simulink model "sm_car_"  (R2026b)
settings: Solver=ode23t  StopTime=100  MaxStep=0.4  AbsTol=1e-3  EnableMultiTasking=on
PreLoadFcn:
  | % Due to usability issue in Repeating Sequence block
  | warning('off','Simulink:Masking:Invalid');
  | 
  | % Eliminate unnecessary warnings in inactive variants
  | % Warnings generated only if you click through inactive variant
  | warning('off','MATLAB:nonExistentField');
  | warning('off','Simulink:Parameters:BlkParamUndefined');
PostLoadFcn:
  | set_param([bdroot '/Vehicle'],'popup_trailer','Off')
  | warning('off','sm:sli:setup:compile:LocalSolverNotSupported')
  | %sm_car_config_maneuver(bdroot,'WOT Braking');
  | sm_car_config_vehicle(bdroot,'false');
  | sm_car_config_logging(bdroot);
InitFcn:
  | sm_car_config_camera;
  | Vehicle = sm_car_vehcfg_checkConfig(Vehicle);
  | sm_car_check_tire_model(bdroot);
StartFcn:
  | tic;
StopFcn:
  | Elapsed_Sim_Time = toc;
  | % disp(['Elapsed Sim Time = ' num2str(Elapsed_Sim_Time)]);
undefined symbols (not defined in the file or in its folder): acc_theta, accel_ramp_rate, Axle1D, AxleIn, Camera, Control, Driver, Init, Maneuver, Pedal, Scene, ShaftL1, ShaftL2, ShaftR1, ShaftR2, Visual, X, xy_data_car_side, Y, Z
libraries: sm_lib x290, fl_lib x171, nesl_utility x144, simulink x60, simulink_extras x14, sdl_lib x14, SimscapeFluids_lib x7, Damper_Element x4, Tire_1x2x x4, ee_lib x3, Scene_Utilities x3, sharedTrackingLibrary x2
(part 21 of 22)

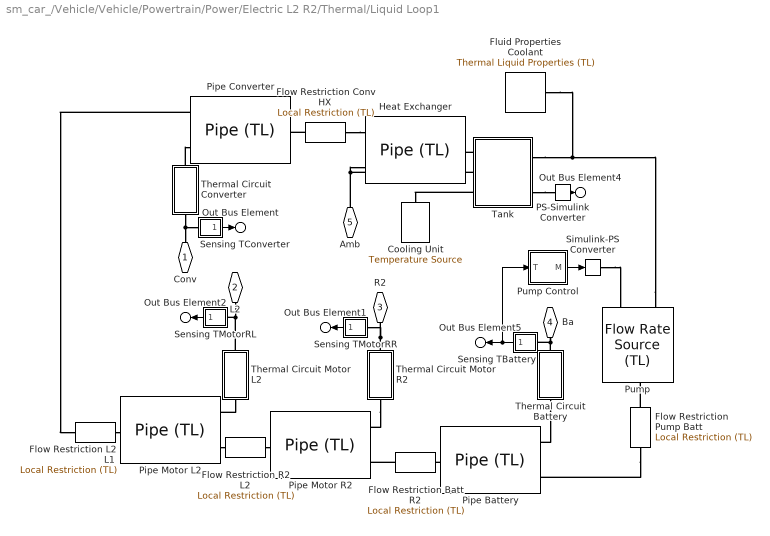
== system sm_car_/Vehicle/Vehicle/Powertrain/Power/Electric L2 R2/Thermal/Liquid Loop1 ==
  Cooling Unit : fl_lib/Thermal/Thermal Sources/Temperature Source  temperature=278 K
  Flow Restriction Batt R2 : fl_lib/Thermal Liquid/Elements/Local Restriction (TL)  restriction_type=foundation.enum.restriction_type.fixed  restriction_area=0.01^2/4*pi*0.5 m^2  min_area=1e-10 m^2  max_area=0.005 m^2  area=0.01^2/4*pi m^2  Cd=0.7  Re_c=12  pressure_recovery=1
  Flow Restriction Conv HX : fl_lib/Thermal Liquid/Elements/Local Restriction (TL)  restriction_type=foundation.enum.restriction_type.fixed  restriction_area=0.01^2/4*pi*0.5 m^2  min_area=1e-10 m^2  max_area=0.005 m^2  area=0.01^2/4*pi m^2  Cd=0.7  Re_c=12  pressure_recovery=1
  Flow Restriction L2 L1 : fl_lib/Thermal Liquid/Elements/Local Restriction (TL)  restriction_type=foundation.enum.restriction_type.fixed  restriction_area=0.01^2/4*pi*0.5 m^2  min_area=1e-10 m^2  max_area=0.005 m^2  area=0.01^2/4*pi m^2  Cd=0.7  Re_c=12  pressure_recovery=1
  Flow Restriction Pump Batt : fl_lib/Thermal Liquid/Elements/Local Restriction (TL)  restriction_type=foundation.enum.restriction_type.fixed  restriction_area=0.01^2/4*pi*0.5 m^2  min_area=1e-10 m^2  max_area=0.005 m^2  area=0.01^2/4*pi m^2  Cd=0.7  Re_c=12  pressure_recovery=1
  Flow Restriction R2 L2 : fl_lib/Thermal Liquid/Elements/Local Restriction (TL)  restriction_type=foundation.enum.restriction_type.fixed  restriction_area=0.01^2/4*pi*0.5 m^2  min_area=1e-10 m^2  max_area=0.005 m^2  area=0.01^2/4*pi m^2  Cd=0.7  Re_c=12  pressure_recovery=1
  "Fluid Properties Coolant " : SimscapeFluids_lib/Thermal Liquid/Utilities/Thermal Liquid Properties (TL)  fluid_list=fluids.thermal_liquid.utilities.enum.thermal_liquid_fluid_list.ethylene_glycol  concentration_param_EG=fluids.thermal_liquid.utilities.enum.thermal_liquid_concentration.volume_fraction  concentration_param_PG=fluids.thermal_liquid.utilities.enum.thermal_liquid_concentration.volume_fraction  c_mass_SW=3.5e-3  c_mass_EG=0.1  c_mass_PG=0.1  c_mass_GL=0.1  c_vol_EG=0.1  c_vol_PG=0.1  beta_const_EG=2.1791 GPa  beta_const_PG=2.1791 GPa  beta_const_GL=2.1791 GPa  p_min_EG=0.01 MPa  p_min_PG=0.01 MPa  p_min_GL=0.01 MPa  p_max_EG=50 MPa  p_max_PG=50 MPa  p_max_GL=50 MPa  T_atm=293.15 K  p_atm=0.101325 MPa  properties_range_check=simscape.enum.assert.action.error  air_fraction=0  R_air=0.287 kJ/(K*kg)  air_dissolution_model=false  p_crit=3 MPa
  Heat Exchanger : SimscapeFluids_lib/Thermal Liquid/Pipes & Fittings/Pipe (TL)  dynamic_compressibility=0  inertia=0  num_segments=1  pipe_length=10 m  cross_section_geometry=fluids.thermal_liquid.pipes_fittings.enum.CrossSectionGeometry.Custom  pipe_diameter=0.1 m  pipe_inner_diameter=0.05 m  pipe_outer_diameter=0.1 m  pipe_width=0.1 m  pipe_height=0.1 m  pipe_major_axis=0.1 m  pipe_minor_axis=0.05 m  pipe_side=0.1 m  pipe_angle=30 deg  area=0.01^2/4*pi m^2  Dh=0.1128 m  annular_heat_transfer_walls=fluids.thermal_liquid.pipes_fittings.enum.AnnularPipeWalls.AnnularInner  elevation_spec=foundation.enum.constant_variable.constant  elevation_gain=0 m  gravity_spec=foundation.enum.constant_variable.constant  g=9.81 m/s^2  pressure_loss_spec=1  local_pressure_loss_spec=fluids.thermal_liquid.pipes_fittings.enum.LocalLossSpec.AggregateLength  length_add=0.1 m  loss_coefficient=0.1  roughness_spec=fluids.thermal_liquid.pipes_fittings.enum.RoughnessSpec.Custom  roughness=1.5e-5 m  Re_friction_TLU=[ 400 1000 1.5e+3 3e+3 4e+3 6e+3 1e+4 2e+4 4e+4 6e+4 1e+5 1e+8 ]  friction_factor_TLU=[ 0.264 0.112 0.07099999999999999 0.0417 0.0387 0.0268 0.025 0.0232 0.0226 0.022 0.0214 0.0214 ]  Re_lam=2e+3  Re_tur=4e+3  shape_factor=64  mdot_nominal=[ 0.1 1 ] kg/s  p_diff_nominal=[ 0.001 0.01 ] MPa  mdot_threshold=1e-6 kg/s  wall_spec=1  vol_expansion_spec=fluids.thermal_liquid.pipes_fittings.enum.VolumeExpansionSpec.Diameter  area_pressure_gain=1e-6 m^2/MPa  static_pressure_TLU=[.1, 1] MPa  area_pressure_gain_TLU=[1e-05, 1.1e-05] m^2  material_behavior_spec=fluids.thermal_liquid.pipes_fittings.enum.PipeMaterialBehavior.Linear  diameter_pressure_gain=1.2e-6 m/MPa  wall_thickness=0.05 m  elastic_modulus=69 GPa  stress_TLU=[276, 310] MPa  strain_TLU=[.004, .02]  stress_assert_action=simscape.enum.assert.action.none  stress_max=400 MPa  poisson_ratio=0.33  wall_time_constant=0.01 s  environment_spec=foundation.enum.pressure_spec.atmospheric  environment_pressure=0.101325 MPa  thermal_expansion=false  alpha_L_wall=24 um/(deltaK*m)  thermal_expansion_Tref=293.15 K  heat_transfer_spec=1  mdot_nominal_heat=[ 0.1 1 ] kg/s  T_in_nominal=[ 293.15 293.15 ] K  T_out_nominal=[ 300 300 ] K  p_in_nominal_heat=[ 0.101325 0.101325 ] MPa  T_wall_nominal=[ 303.15 303.15 ] K  T_wall_eff_nominal=[303.15, 303.15] K  a_coeff=0.023  b_Re_power=0.8  c_Pr_power=0.4  Nu_lam=3.66  Re_Colburn_TLU=[ 100 150 1000 ]  Colburn_factor_TLU=[ 0.019 0.013 0.002 ]  Re_Nu_TLU=[ 100 150 1000 ]  Pr_Nu_TLU=[ 1 10 ]  Nu_TLU=[ 3.72 4.21; 3.75 4.44; 4.21 7.15 ]  annular_correction=fluids.thermal_liquid.pipes_fittings.enum.AnnularPipeCorrectionFactor.Gnielinski  p0_vec=0.101325 MPa  T0_vec=300 K  mdot0=0.1 kg/s  p_nominal=0.101325 MPa  T_nominal=293.15 K
  PS-Simulink Converter : nesl_utility/PS-Simulink Converter  PhysicalDomain=network_engine_domain  SubClassName=ps_output  LeftPortType=input  RightPortType=output  PseudoPeriodic=off  Frequencies=[]  VectorFormat=1-D array  Unit=1  AffineConversion=off
  Pipe Battery : SimscapeFluids_lib/Thermal Liquid/Pipes & Fittings/Pipe (TL)  dynamic_compressibility=0  inertia=0  num_segments=1  pipe_length=1 m  cross_section_geometry=fluids.thermal_liquid.pipes_fittings.enum.CrossSectionGeometry.Custom  pipe_diameter=0.1 m  pipe_inner_diameter=0.05 m  pipe_outer_diameter=0.1 m  pipe_width=0.1 m  pipe_height=0.1 m  pipe_major_axis=0.1 m  pipe_minor_axis=0.05 m  pipe_side=0.1 m  pipe_angle=30 deg  area=0.01^2/4*pi m^2  Dh=0.1128 m  annular_heat_transfer_walls=fluids.thermal_liquid.pipes_fittings.enum.AnnularPipeWalls.AnnularInner  elevation_spec=foundation.enum.constant_variable.constant  elevation_gain=0 m  gravity_spec=foundation.enum.constant_variable.constant  g=9.81 m/s^2  pressure_loss_spec=1  local_pressure_loss_spec=fluids.thermal_liquid.pipes_fittings.enum.LocalLossSpec.AggregateLength  length_add=0.1 m  loss_coefficient=0.1  roughness_spec=fluids.thermal_liquid.pipes_fittings.enum.RoughnessSpec.Custom  roughness=1.5e-5 m  Re_friction_TLU=[ 400 1000 1.5e+3 3e+3 4e+3 6e+3 1e+4 2e+4 4e+4 6e+4 1e+5 1e+8 ]  friction_factor_TLU=[ 0.264 0.112 0.07099999999999999 0.0417 0.0387 0.0268 0.025 0.0232 0.0226 0.022 0.0214 0.0214 ]  Re_lam=2e+3  Re_tur=4e+3  shape_factor=64  mdot_nominal=[ 0.1 1 ] kg/s  p_diff_nominal=[ 0.001 0.01 ] MPa  mdot_threshold=1e-6 kg/s  wall_spec=1  vol_expansion_spec=fluids.thermal_liquid.pipes_fittings.enum.VolumeExpansionSpec.Diameter  area_pressure_gain=1e-6 m^2/MPa  static_pressure_TLU=[.1, 1] MPa  area_pressure_gain_TLU=[1e-05, 1.1e-05] m^2  material_behavior_spec=fluids.thermal_liquid.pipes_fittings.enum.PipeMaterialBehavior.Linear  diameter_pressure_gain=1.2e-6 m/MPa  wall_thickness=0.05 m  elastic_modulus=69 GPa  stress_TLU=[276, 310] MPa  strain_TLU=[.004, .02]  stress_assert_action=simscape.enum.assert.action.none  stress_max=400 MPa  poisson_ratio=0.33  wall_time_constant=0.01 s  environment_spec=foundation.enum.pressure_spec.atmospheric  environment_pressure=0.101325 MPa  thermal_expansion=false  alpha_L_wall=24 um/(deltaK*m)  thermal_expansion_Tref=293.15 K  heat_transfer_spec=1  mdot_nominal_heat=[ 0.1 1 ] kg/s  T_in_nominal=[ 293.15 293.15 ] K  T_out_nominal=[ 300 300 ] K  p_in_nominal_heat=[ 0.101325 0.101325 ] MPa  T_wall_nominal=[ 303.15 303.15 ] K  T_wall_eff_nominal=[303.15, 303.15] K  a_coeff=0.023  b_Re_power=0.8  c_Pr_power=0.4  Nu_lam=3.66  Re_Colburn_TLU=[ 100 150 1000 ]  Colburn_factor_TLU=[ 0.019 0.013 0.002 ]  Re_Nu_TLU=[ 100 150 1000 ]  Pr_Nu_TLU=[ 1 10 ]  Nu_TLU=[ 3.72 4.21; 3.75 4.44; 4.21 7.15 ]  annular_correction=fluids.thermal_liquid.pipes_fittings.enum.AnnularPipeCorrectionFactor.Gnielinski  p0_vec=0.101325 MPa  T0_vec=300 K  mdot0=0.1 kg/s  p_nominal=0.101325 MPa  T_nominal=293.15 K
  Pipe Converter : SimscapeFluids_lib/Thermal Liquid/Pipes & Fittings/Pipe (TL)  dynamic_compressibility=0  inertia=0  num_segments=1  pipe_length=1 m  cross_section_geometry=fluids.thermal_liquid.pipes_fittings.enum.CrossSectionGeometry.Custom  pipe_diameter=0.1 m  pipe_inner_diameter=0.05 m  pipe_outer_diameter=0.1 m  pipe_width=0.1 m  pipe_height=0.1 m  pipe_major_axis=0.1 m  pipe_minor_axis=0.05 m  pipe_side=0.1 m  pipe_angle=30 deg  area=0.01^2/4*pi m^2  Dh=0.1128 m  annular_heat_transfer_walls=fluids.thermal_liquid.pipes_fittings.enum.AnnularPipeWalls.AnnularInner  elevation_spec=foundation.enum.constant_variable.constant  elevation_gain=0 m  gravity_spec=foundation.enum.constant_variable.constant  g=9.81 m/s^2  pressure_loss_spec=1  local_pressure_loss_spec=fluids.thermal_liquid.pipes_fittings.enum.LocalLossSpec.AggregateLength  length_add=0.1 m  loss_coefficient=0.1  roughness_spec=fluids.thermal_liquid.pipes_fittings.enum.RoughnessSpec.Custom  roughness=1.5e-5 m  Re_friction_TLU=[ 400 1000 1.5e+3 3e+3 4e+3 6e+3 1e+4 2e+4 4e+4 6e+4 1e+5 1e+8 ]  friction_factor_TLU=[ 0.264 0.112 0.07099999999999999 0.0417 0.0387 0.0268 0.025 0.0232 0.0226 0.022 0.0214 0.0214 ]  Re_lam=2e+3  Re_tur=4e+3  shape_factor=64  mdot_nominal=[ 0.1 1 ] kg/s  p_diff_nominal=[ 0.001 0.01 ] MPa  mdot_threshold=1e-6 kg/s  wall_spec=1  vol_expansion_spec=fluids.thermal_liquid.pipes_fittings.enum.VolumeExpansionSpec.Diameter  area_pressure_gain=1e-6 m^2/MPa  static_pressure_TLU=[.1, 1] MPa  area_pressure_gain_TLU=[1e-05, 1.1e-05] m^2  material_behavior_spec=fluids.thermal_liquid.pipes_fittings.enum.PipeMaterialBehavior.Linear  diameter_pressure_gain=1.2e-6 m/MPa  wall_thickness=0.05 m  elastic_modulus=69 GPa  stress_TLU=[276, 310] MPa  strain_TLU=[.004, .02]  stress_assert_action=simscape.enum.assert.action.none  stress_max=400 MPa  poisson_ratio=0.33  wall_time_constant=0.01 s  environment_spec=foundation.enum.pressure_spec.atmospheric  environment_pressure=0.101325 MPa  thermal_expansion=false  alpha_L_wall=24 um/(deltaK*m)  thermal_expansion_Tref=293.15 K  heat_transfer_spec=1  mdot_nominal_heat=[ 0.1 1 ] kg/s  T_in_nominal=[ 293.15 293.15 ] K  T_out_nominal=[ 300 300 ] K  p_in_nominal_heat=[ 0.101325 0.101325 ] MPa  T_wall_nominal=[ 303.15 303.15 ] K  T_wall_eff_nominal=[303.15, 303.15] K  a_coeff=0.023  b_Re_power=0.8  c_Pr_power=0.4  Nu_lam=3.66  Re_Colburn_TLU=[ 100 150 1000 ]  Colburn_factor_TLU=[ 0.019 0.013 0.002 ]  Re_Nu_TLU=[ 100 150 1000 ]  Pr_Nu_TLU=[ 1 10 ]  Nu_TLU=[ 3.72 4.21; 3.75 4.44; 4.21 7.15 ]  annular_correction=fluids.thermal_liquid.pipes_fittings.enum.AnnularPipeCorrectionFactor.Gnielinski  p0_vec=0.101325 MPa  T0_vec=300 K  mdot0=0.1 kg/s  p_nominal=0.101325 MPa  T_nominal=293.15 K
  Pipe Motor L2 : SimscapeFluids_lib/Thermal Liquid/Pipes & Fittings/Pipe (TL)  dynamic_compressibility=0  inertia=0  num_segments=1  pipe_length=1 m  cross_section_geometry=fluids.thermal_liquid.pipes_fittings.enum.CrossSectionGeometry.Custom  pipe_diameter=0.1 m  pipe_inner_diameter=0.05 m  pipe_outer_diameter=0.1 m  pipe_width=0.1 m  pipe_height=0.1 m  pipe_major_axis=0.1 m  pipe_minor_axis=0.05 m  pipe_side=0.1 m  pipe_angle=30 deg  area=0.01^2/4*pi m^2  Dh=0.1128 m  annular_heat_transfer_walls=fluids.thermal_liquid.pipes_fittings.enum.AnnularPipeWalls.AnnularInner  elevation_spec=foundation.enum.constant_variable.constant  elevation_gain=0 m  gravity_spec=foundation.enum.constant_variable.constant  g=9.81 m/s^2  pressure_loss_spec=1  local_pressure_loss_spec=fluids.thermal_liquid.pipes_fittings.enum.LocalLossSpec.AggregateLength  length_add=0.1 m  loss_coefficient=0.1  roughness_spec=fluids.thermal_liquid.pipes_fittings.enum.RoughnessSpec.Custom  roughness=1.5e-5 m  Re_friction_TLU=[ 400 1000 1.5e+3 3e+3 4e+3 6e+3 1e+4 2e+4 4e+4 6e+4 1e+5 1e+8 ]  friction_factor_TLU=[ 0.264 0.112 0.07099999999999999 0.0417 0.0387 0.0268 0.025 0.0232 0.0226 0.022 0.0214 0.0214 ]  Re_lam=2e+3  Re_tur=4e+3  shape_factor=64  mdot_nominal=[ 0.1 1 ] kg/s  p_diff_nominal=[ 0.001 0.01 ] MPa  mdot_threshold=1e-6 kg/s  wall_spec=1  vol_expansion_spec=fluids.thermal_liquid.pipes_fittings.enum.VolumeExpansionSpec.Diameter  area_pressure_gain=1e-6 m^2/MPa  static_pressure_TLU=[.1, 1] MPa  area_pressure_gain_TLU=[1e-05, 1.1e-05] m^2  material_behavior_spec=fluids.thermal_liquid.pipes_fittings.enum.PipeMaterialBehavior.Linear  diameter_pressure_gain=1.2e-6 m/MPa  wall_thickness=0.05 m  elastic_modulus=69 GPa  stress_TLU=[276, 310] MPa  strain_TLU=[.004, .02]  stress_assert_action=simscape.enum.assert.action.none  stress_max=400 MPa  poisson_ratio=0.33  wall_time_constant=0.01 s  environment_spec=foundation.enum.pressure_spec.atmospheric  environment_pressure=0.101325 MPa  thermal_expansion=false  alpha_L_wall=24 um/(deltaK*m)  thermal_expansion_Tref=293.15 K  heat_transfer_spec=1  mdot_nominal_heat=[ 0.1 1 ] kg/s  T_in_nominal=[ 293.15 293.15 ] K  T_out_nominal=[ 300 300 ] K  p_in_nominal_heat=[ 0.101325 0.101325 ] MPa  T_wall_nominal=[ 303.15 303.15 ] K  T_wall_eff_nominal=[303.15, 303.15] K  a_coeff=0.023  b_Re_power=0.8  c_Pr_power=0.4  Nu_lam=3.66  Re_Colburn_TLU=[ 100 150 1000 ]  Colburn_factor_TLU=[ 0.019 0.013 0.002 ]  Re_Nu_TLU=[ 100 150 1000 ]  Pr_Nu_TLU=[ 1 10 ]  Nu_TLU=[ 3.72 4.21; 3.75 4.44; 4.21 7.15 ]  annular_correction=fluids.thermal_liquid.pipes_fittings.enum.AnnularPipeCorrectionFactor.Gnielinski  p0_vec=0.101325 MPa  T0_vec=300 K  mdot0=0.1 kg/s  p_nominal=0.101325 MPa  T_nominal=293.15 K
  Pipe Motor R2 : SimscapeFluids_lib/Thermal Liquid/Pipes & Fittings/Pipe (TL)  dynamic_compressibility=0  inertia=0  num_segments=1  pipe_length=1 m  cross_section_geometry=fluids.thermal_liquid.pipes_fittings.enum.CrossSectionGeometry.Custom  pipe_diameter=0.1 m  pipe_inner_diameter=0.05 m  pipe_outer_diameter=0.1 m  pipe_width=0.1 m  pipe_height=0.1 m  pipe_major_axis=0.1 m  pipe_minor_axis=0.05 m  pipe_side=0.1 m  pipe_angle=30 deg  area=0.01^2/4*pi m^2  Dh=0.1128 m  annular_heat_transfer_walls=fluids.thermal_liquid.pipes_fittings.enum.AnnularPipeWalls.AnnularInner  elevation_spec=foundation.enum.constant_variable.constant  elevation_gain=0 m  gravity_spec=foundation.enum.constant_variable.constant  g=9.81 m/s^2  pressure_loss_spec=1  local_pressure_loss_spec=fluids.thermal_liquid.pipes_fittings.enum.LocalLossSpec.AggregateLength  length_add=0.1 m  loss_coefficient=0.1  roughness_spec=fluids.thermal_liquid.pipes_fittings.enum.RoughnessSpec.Custom  roughness=1.5e-5 m  Re_friction_TLU=[ 400 1000 1.5e+3 3e+3 4e+3 6e+3 1e+4 2e+4 4e+4 6e+4 1e+5 1e+8 ]  friction_factor_TLU=[ 0.264 0.112 0.07099999999999999 0.0417 0.0387 0.0268 0.025 0.0232 0.0226 0.022 0.0214 0.0214 ]  Re_lam=2e+3  Re_tur=4e+3  shape_factor=64  mdot_nominal=[ 0.1 1 ] kg/s  p_diff_nominal=[ 0.001 0.01 ] MPa  mdot_threshold=1e-6 kg/s  wall_spec=1  vol_expansion_spec=fluids.thermal_liquid.pipes_fittings.enum.VolumeExpansionSpec.Diameter  area_pressure_gain=1e-6 m^2/MPa  static_pressure_TLU=[.1, 1] MPa  area_pressure_gain_TLU=[1e-05, 1.1e-05] m^2  material_behavior_spec=fluids.thermal_liquid.pipes_fittings.enum.PipeMaterialBehavior.Linear  diameter_pressure_gain=1.2e-6 m/MPa  wall_thickness=0.05 m  elastic_modulus=69 GPa  stress_TLU=[276, 310] MPa  strain_TLU=[.004, .02]  stress_assert_action=simscape.enum.assert.action.none  stress_max=400 MPa  poisson_ratio=0.33  wall_time_constant=0.01 s  environment_spec=foundation.enum.pressure_spec.atmospheric  environment_pressure=0.101325 MPa  thermal_expansion=false  alpha_L_wall=24 um/(deltaK*m)  thermal_expansion_Tref=293.15 K  heat_transfer_spec=1  mdot_nominal_heat=[ 0.1 1 ] kg/s  T_in_nominal=[ 293.15 293.15 ] K  T_out_nominal=[ 300 300 ] K  p_in_nominal_heat=[ 0.101325 0.101325 ] MPa  T_wall_nominal=[ 303.15 303.15 ] K  T_wall_eff_nominal=[303.15, 303.15] K  a_coeff=0.023  b_Re_power=0.8  c_Pr_power=0.4  Nu_lam=3.66  Re_Colburn_TLU=[ 100 150 1000 ]  Colburn_factor_TLU=[ 0.019 0.013 0.002 ]  Re_Nu_TLU=[ 100 150 1000 ]  Pr_Nu_TLU=[ 1 10 ]  Nu_TLU=[ 3.72 4.21; 3.75 4.44; 4.21 7.15 ]  annular_correction=fluids.thermal_liquid.pipes_fittings.enum.AnnularPipeCorrectionFactor.Gnielinski  p0_vec=0.101325 MPa  T0_vec=300 K  mdot0=0.1 kg/s  p_nominal=0.101325 MPa  T_nominal=293.15 K
  Pump : fl_lib/Thermal Liquid/Sources/Flow Rate Source (TL)  source_type=foundation.enum.constant_controlled.controlled  flow_type=foundation.enum.mass_volumetric_flow.mass  mass_flow=0 kg/s  volumetric_flow=0 m^3/s  power_spec=foundation.enum.power_spec.isentropic  area=0.01^2/4*pi m^2
  Pump Control : Subsystem
  Sensing TBattery : Subsystem
  Sensing TConverter : Subsystem
  Sensing TMotorRL : Subsystem
  Sensing TMotorRR : Subsystem
  Simulink-PS Converter : nesl_utility/Simulink-PS Converter  PhysicalDomain=network_engine_domain  SubClassName=ps_input  LeftPortType=input  RightPortType=output  PseudoPeriodic=off  Frequencies=[]  NoiseDistribution=none  NoiseParameters=[]  Unit=kg/s  AffineConversion=off  FilteringAndDerivatives=provide  SimscapeFilterOrder=1  InputFilterTimeConstant=0.001  UdotUserProvided=0
  Tank : Subsystem
  Thermal Circuit Battery : Subsystem
  Thermal Circuit Converter : Subsystem
  Thermal Circuit Motor L2 : Subsystem
  Thermal Circuit Motor R2 : Subsystem
  Conv : PMIOPort  Side=Left
  L2 : PMIOPort  Port=2  Side=Left
  R2 : PMIOPort  Port=3  Side=Left
  Ba : PMIOPort  Port=4  Side=Right
  Amb : PMIOPort  Port=5  Side=Right
  Out Bus Element : Outport  VectorParamsAs1DForOutWhenUnconnected=off  PortName=m  Element=TConverter
  Out Bus Element1 : Outport  VectorParamsAs1DForOutWhenUnconnected=off  PortName=m  Element=TMotorR2
  Out Bus Element2 : Outport  VectorParamsAs1DForOutWhenUnconnected=off  PortName=m  Element=TMotorL2
  Out Bus Element4 : Outport  VectorParamsAs1DForOutWhenUnconnected=off  PortName=m  Element=TCoolant
  Out Bus Element5 : Outport  VectorParamsAs1DForOutWhenUnconnected=off  PortName=m  Element=TBattery
  wires:
  Sensing TBattery/1(T) -> Pump Control/1(T), Out Bus Element5/1
  PS-Simulink Converter/1 -> Out Bus Element4/1
  Sensing TMotorRL/1(T) -> Out Bus Element2/1
  Sensing TConverter/1(T) -> Out Bus Element/1
  Pump Control/1(M) -> Simulink-PS Converter/1
  Sensing TMotorRR/1(T) -> Out Bus Element1/1
  connections:
  Flow Restriction L2 L1/LConn1 -- Pipe Motor L2/RConn1
  Tank/LConn3 -- Cooling Unit/LConn1
  Thermal Circuit Battery/RConn1 -- Pipe Battery/LConn2
  Sensing TBattery/LConn1 -- Thermal Circuit Battery/LConn1 -- Ba/RConn1
  Thermal Circuit Converter/RConn1 -- Pipe Converter/LConn2
  Flow Restriction Conv HX/LConn1 -- Pipe Converter/RConn1
  Pipe Converter/LConn1 -- Flow Restriction L2 L1/RConn1
  Tank/RConn2 -- PS-Simulink Converter/LConn1
  Pump/LConn1 -- Tank/RConn1 -- "Fluid Properties Coolant "/RConn1
  Tank/LConn1 -- Heat Exchanger/RConn1
  Heat Exchanger/LConn2 -- Tank/LConn2 -- Amb/RConn1
  Flow Restriction Conv HX/RConn1 -- Heat Exchanger/LConn1
  Flow Restriction Batt R2/RConn1 -- Pipe Motor R2/LConn1
  Pipe Battery/RConn1 -- Flow Restriction Batt R2/LConn1
  Flow Restriction Pump Batt/LConn1 -- Pump/RConn1
  Simulink-PS Converter/RConn1 -- Pump/LConn2
  R2/RConn1 -- Thermal Circuit Motor R2/LConn1 -- Sensing TMotorRR/LConn1
  Flow Restriction Pump Batt/RConn1 -- Pipe Battery/LConn1
  Conv/RConn1 -- Thermal Circuit Converter/LConn1 -- Sensing TConverter/LConn1
  Thermal Circuit Motor R2/RConn1 -- Pipe Motor R2/LConn2
  Thermal Circuit Motor L2/LConn1 -- Sensing TMotorRL/LConn1 -- L2/RConn1
  Thermal Circuit Motor L2/RConn1 -- Pipe Motor L2/LConn2
  Pipe Motor L2/LConn1 -- Flow Restriction R2 L2/RConn1
  Flow Restriction R2 L2/LConn1 -- Pipe Motor R2/RConn1

== system sm_car_/Vehicle/Vehicle/Powertrain/Power/Electric L2 R2/Thermal/Liquid Loop1/Pump Control ==
  T : Inport
  Memory : Memory
  Pump Time Constant : TransferFcn  Denominator=[0.1 1]
  Relay : Relay  OnSwitchValue=313  OffSwitchValue=293  ZeroCross=off
  M : Outport  VectorParamsAs1DForOutWhenUnconnected=off
  wires:
  Pump Time Constant/1 -> M/1
  Memory/1 -> Relay/1
  T/1 -> Memory/1
  Relay/1 -> Pump Time Constant/1  "Pump_flw"

== system sm_car_/Vehicle/Vehicle/Powertrain/Power/Electric L2 R2/Thermal/Liquid Loop1/Sensing TBattery ==
  PS-Simulink Converter4 : nesl_utility/PS-Simulink Converter  PhysicalDomain=network_engine_domain  SubClassName=ps_output  LeftPortType=input  RightPortType=output  PseudoPeriodic=off  Frequencies=[]  VectorFormat=1-D array  Unit=K  AffineConversion=on
  Temperature Sensor : fl_lib/Thermal/Thermal Sensors/Temperature Sensor  temperature_measure=foundation.enum.MeasurementReference.difference
  Thermal Reference : fl_lib/Thermal/Thermal Elements/Thermal Reference
  A : PMIOPort  Side=Left
  T : Outport  VectorParamsAs1DForOutWhenUnconnected=off
  wires:
  PS-Simulink Converter4/1 -> T/1  "Temperature"
  connections:
  Temperature Sensor/LConn1 -- A/RConn1
  Thermal Reference/LConn1 -- Temperature Sensor/RConn1
  Temperature Sensor/RConn2 -- PS-Simulink Converter4/LConn1

== system sm_car_/Vehicle/Vehicle/Powertrain/Power/Electric L2 R2/Thermal/Liquid Loop1/Sensing TConverter ==
  PS-Simulink Converter4 : nesl_utility/PS-Simulink Converter  PhysicalDomain=network_engine_domain  SubClassName=ps_output  LeftPortType=input  RightPortType=output  PseudoPeriodic=off  Frequencies=[]  VectorFormat=1-D array  Unit=K  AffineConversion=on
  Temperature Sensor : fl_lib/Thermal/Thermal Sensors/Temperature Sensor  temperature_measure=foundation.enum.MeasurementReference.difference
  Thermal Reference : fl_lib/Thermal/Thermal Elements/Thermal Reference
  A : PMIOPort  Side=Left
  T : Outport  VectorParamsAs1DForOutWhenUnconnected=off
  wires:
  PS-Simulink Converter4/1 -> T/1  "Temperature"
  connections:
  Temperature Sensor/RConn2 -- PS-Simulink Converter4/LConn1
  Thermal Reference/LConn1 -- Temperature Sensor/RConn1
  Temperature Sensor/LConn1 -- A/RConn1

== system sm_car_/Vehicle/Vehicle/Powertrain/Power/Electric L2 R2/Thermal/Liquid Loop1/Sensing TMotorRL ==
  PS-Simulink Converter4 : nesl_utility/PS-Simulink Converter  PhysicalDomain=network_engine_domain  SubClassName=ps_output  LeftPortType=input  RightPortType=output  PseudoPeriodic=off  Frequencies=[]  VectorFormat=1-D array  Unit=K  AffineConversion=on
  Temperature Sensor : fl_lib/Thermal/Thermal Sensors/Temperature Sensor  temperature_measure=foundation.enum.MeasurementReference.difference
  Thermal Reference : fl_lib/Thermal/Thermal Elements/Thermal Reference
  A : PMIOPort  Side=Left
  T : Outport  VectorParamsAs1DForOutWhenUnconnected=off
  wires:
  PS-Simulink Converter4/1 -> T/1  "Temperature"
  connections:
  Temperature Sensor/LConn1 -- A/RConn1
  Thermal Reference/LConn1 -- Temperature Sensor/RConn1
  Temperature Sensor/RConn2 -- PS-Simulink Converter4/LConn1

== system sm_car_/Vehicle/Vehicle/Powertrain/Power/Electric L2 R2/Thermal/Liquid Loop1/Sensing TMotorRR ==
  PS-Simulink Converter4 : nesl_utility/PS-Simulink Converter  PhysicalDomain=network_engine_domain  SubClassName=ps_output  LeftPortType=input  RightPortType=output  PseudoPeriodic=off  Frequencies=[]  VectorFormat=1-D array  Unit=K  AffineConversion=on
  Temperature Sensor : fl_lib/Thermal/Thermal Sensors/Temperature Sensor  temperature_measure=foundation.enum.MeasurementReference.difference
  Thermal Reference : fl_lib/Thermal/Thermal Elements/Thermal Reference
  A : PMIOPort  Side=Left
  T : Outport  VectorParamsAs1DForOutWhenUnconnected=off
  wires:
  PS-Simulink Converter4/1 -> T/1  "Temperature"
  connections:
  Temperature Sensor/LConn1 -- A/RConn1
  Thermal Reference/LConn1 -- Temperature Sensor/RConn1
  Temperature Sensor/RConn2 -- PS-Simulink Converter4/LConn1

== system sm_car_/Vehicle/Vehicle/Powertrain/Power/Electric L2 R2/Thermal/Liquid Loop1/Tank ==
  Absolute Reference (TL) : fl_lib/Thermal Liquid/Elements/Absolute Reference (TL)
  Cap (G) : fl_lib/Gas/Elements/Cap (G)  p_specify=off  p_priority=None  p=0.101325 MPa  p_nominal_specify=off  p_nominal_value=1  p_nominal_unit=MPa  T_specify=off  T_priority=None  T=293.15 K  T_nominal_specify=off  T_nominal_value=1  T_nominal_unit=K
  Convective Heat Transfer : fl_lib/Thermal/Thermal Elements/Convective Heat Transfer  thermal_type=foundation.enum.constant_variable.constant  area=1 m^2  heat_tr_coeff=20 W/(m^2 * K)  min_heat_tr_coeff=1e-3 W/(K*m^2)  T_specify=off  T_priority=None  T=0 K  T_nominal_specify=off  T_nominal_value=1  T_nominal_unit=K  Q_specify=off  Q_priority=None  Q=0 W  Q_nominal_specify=off  Q_nominal_value=1  Q_nominal_unit=W
  Convective Heat Transfer1 : fl_lib/Thermal/Thermal Elements/Convective Heat Transfer  thermal_type=foundation.enum.constant_variable.constant  area=1 m^2  heat_tr_coeff=200 W/(m^2 * K)  min_heat_tr_coeff=1e-3 W/(K*m^2)  T_specify=off  T_priority=None  T=0 K  T_nominal_specify=off  T_nominal_value=1  T_nominal_unit=K  Q_specify=off  Q_priority=None  Q=0 W  Q_nominal_specify=off  Q_nominal_value=1  Q_nominal_unit=W
  PS Terminator : fl_lib/Physical Signals/Sinks/PS Terminator
  PS Terminator1 : fl_lib/Physical Signals/Sinks/PS Terminator
  PS Terminator2 : fl_lib/Physical Signals/Sinks/PS Terminator
  Reservoir (G) : fl_lib/Gas/Elements/Reservoir (G)  reservoir_spec=foundation.enum.ReservoirSpec.StaticPressureTemperature  pressure_input=false  pressure_spec=1  reservoir_pressure=0.101325 MPa  temperature_input=false  reservoir_temperature=25 degC  area_A=0.001 m^2  input_error_spec=foundation.enum.input_range_error.warn
  Sensor P T : fl_lib/Thermal Liquid/Sensors/Pressure & Temperature Sensor (TL)  reference=foundation.enum.MeasurementReference.difference  pressure=true  pressure_spec=foundation.enum.PressureMeasementSpec.Absolute  temperature=true
  Tank : SimscapeFluids_lib/Thermal Liquid/Tanks & Accumulators/Tank (G-TL)  num_inlet=2  volume_total=0.01 m^3  volume_spec=1  tank_area=0.005 m^2  level_TLU=[0, 3, 5] m  volume_TLU=[0, 4, 6] m^3  inlet_areas_A1B1=[.001, .001] m^2  inlet_height_A2=0.1 m  inlet_area_A2=0.01 m^2  inlet_heights_A2B2=[.01, 0.01] m  inlet_areas_A2B2=[0.01^2/4*pi, 0.01^2/4*pi] m^2  inlet_heights_A2B2C2=[.1, .1, .1] m  inlet_areas_A2B2C2=[.01, .01, .01] m^2  inlet_heights_A2B2C2D2=0.1 * ones(1, 4) m  inlet_areas_A2B2C2D2=0.01 * ones(1, 4) m^2  inlet_heights_A2B2C2D2E2=0.1 * ones(1, 5) m  inlet_areas_A2B2C2D2E2=0.01 * ones(1, 5) m^2  inlet_heights_A2B2C2D2E2F2=0.1 * ones(1, 6) m  inlet_areas_A2B2C2D2E2F2=0.01 * ones(1, 6) m^2  capacity_check=0  max_liquid_capacity=0.01 m^3  g=9.81 m/s^2  level_specify=on  level_priority=High  level=0.1 m  level_nominal_specify=off  level_nominal_value=1  level_nominal_unit=m  volume_liquid_specify=off  volume_liquid_priority=None  volume_liquid=5 m^3  volume_liquid_nominal_specify=off  volume_liquid_nominal_value=1  volume_liquid_nominal_unit=m^3  mass_liquid_specify=off  mass_liquid_priority=None  mass_liquid=5e+3 kg  mass_liquid_nominal_specify=off  mass_liquid_nominal_value=1  mass_liquid_nominal_unit=kg  T_liquid_specify=on  T_liquid_priority=High  T_liquid=278 K  T_liquid_nominal_specify=off  T_liquid_nominal_value=1  T_liquid_nominal_unit=K  p_gas_specify=off  p_gas_priority=High  p_gas=0.101325 MPa  p_gas_nominal_specify=off  p_gas_nominal_value=1  p_gas_nominal_unit=MPa  T_gas_specify=on  T_gas_priority=High  T_gas=278 K  T_gas_nominal_specify=off  T_gas_nominal_value=1  T_gas_nominal_unit=K  rho_gas_specify=off  rho_gas_priority=None  rho_gas=1.2 kg/m^3  rho_gas_nominal_specify=off  rho_gas_nominal_value=1  rho_gas_nominal_unit=kg/m^3
  B : PMIOPort  Side=Left
  HGas : PMIOPort  Port=2  Side=Left
  A : PMIOPort  Port=3  Side=Right
  T : PMIOPort  Port=4  Side=Right
  HLiq : PMIOPort  Port=5  Side=Left
  connections:
  Tank/LConn6 -- PS Terminator1/LConn1
  Tank/LConn5 -- PS Terminator/LConn1
  HLiq/RConn1 -- Convective Heat Transfer1/RConn1
  Convective Heat Transfer/LConn1 -- Tank/RConn1
  HGas/RConn1 -- Convective Heat Transfer/RConn1
  Sensor P T/RConn2 -- PS Terminator2/LConn1
  Cap (G)/LConn1 -- Tank/LConn2
  Tank/LConn3 -- A/RConn1
  Reservoir (G)/LConn1 -- Tank/LConn1
  Absolute Reference (TL)/LConn1 -- Sensor P T/RConn1
  Sensor P T/RConn3 -- T/RConn1
  Tank/LConn4 -- B/RConn1 -- Sensor P T/LConn1
  Convective Heat Transfer1/LConn1 -- Tank/RConn2

== system sm_car_/Vehicle/Vehicle/Powertrain/Power/Electric L2 R2/Thermal/Liquid Loop1/Thermal Circuit Battery ==
  Conductive Heat Transfer : fl_lib/Thermal/Thermal Elements/Conductive Heat Transfer  thermal_type=foundation.enum.ConstantVariableTabulated.Constant  wall_geometry=foundation.enum.ConductionWallGeometry.Planar  area=pi m^2  thickness=0.004 m  d_in=0.05 m  d_out=0.1 m  L=1 m  th_cond_min=10 W/(K*m)  th_cond="237;  %Al W/(m*K)"  th_cond_TLU=[413, 401, 392, 383, 371, 357, 342] W/(K*m)  temp_TLU=[200, 273, 400, 600, 800, 1000, 1200] K  T_specify=off  T_priority=None  T=0 K  T_nominal_specify=off  T_nominal_value=1  T_nominal_unit=K  Q_specify=off  Q_priority=None  Q=0 W  Q_nominal_specify=off  Q_nominal_value=1  Q_nominal_unit=W
  Thermal Mass : fl_lib/Thermal/Thermal Elements/Thermal Mass  mass_type=foundation.enum.constant_variable.constant  mass=2 kg  sp_heat=910 J/kg/K  mass_min=1e-6 kg  num_ports=foundation.enum.numPorts2.one  m_specify=off  m_priority=High  m=1 kg  m_nominal_specify=off  m_nominal_value=1  m_nominal_unit=kg  T_specify=off  T_priority=High  T=300 K  T_nominal_specify=off  T_nominal_value=1  T_nominal_unit=K  Q_specify=off  Q_priority=None  Q=0 W  Q_nominal_specify=off  Q_nominal_value=1  Q_nominal_unit=W
  A : PMIOPort  Side=Left
  B : PMIOPort  Port=2  Side=Right
  connections:
  A/RConn1 -- Conductive Heat Transfer/LConn1
  Conductive Heat Transfer/RConn1 -- B/RConn1 -- Thermal Mass/LConn1

== system sm_car_/Vehicle/Vehicle/Powertrain/Power/Electric L2 R2/Thermal/Liquid Loop1/Thermal Circuit Converter ==
  Conductive Heat Transfer : fl_lib/Thermal/Thermal Elements/Conductive Heat Transfer  thermal_type=foundation.enum.ConstantVariableTabulated.Constant  wall_geometry=foundation.enum.ConductionWallGeometry.Planar  area=0.01*pi*1 m^2  thickness=0.004 m  d_in=0.05 m  d_out=0.1 m  L=1 m  th_cond_min=10 W/(K*m)  th_cond="237;  %Al W/(m*K)"  th_cond_TLU=[413, 401, 392, 383, 371, 357, 342] W/(K*m)  temp_TLU=[200, 273, 400, 600, 800, 1000, 1200] K  T_specify=off  T_priority=None  T=0 K  T_nominal_specify=off  T_nominal_value=1  T_nominal_unit=K  Q_specify=off  Q_priority=None  Q=0 W  Q_nominal_specify=off  Q_nominal_value=1  Q_nominal_unit=W
  Thermal Mass : fl_lib/Thermal/Thermal Elements/Thermal Mass  mass_type=foundation.enum.constant_variable.constant  mass=2 kg  sp_heat=910 J/kg/K  mass_min=1e-6 kg  num_ports=foundation.enum.numPorts2.one  m_specify=off  m_priority=High  m=1 kg  m_nominal_specify=off  m_nominal_value=1  m_nominal_unit=kg  T_specify=off  T_priority=High  T=300 K  T_nominal_specify=off  T_nominal_value=1  T_nominal_unit=K  Q_specify=off  Q_priority=None  Q=0 W  Q_nominal_specify=off  Q_nominal_value=1  Q_nominal_unit=W
  A : PMIOPort  Side=Left
  B : PMIOPort  Port=2  Side=Right
  connections:
  A/RConn1 -- Conductive Heat Transfer/LConn1
  B/RConn1 -- Conductive Heat Transfer/RConn1 -- Thermal Mass/LConn1

== system sm_car_/Vehicle/Vehicle/Powertrain/Power/Electric L2 R2/Thermal/Liquid Loop1/Thermal Circuit Motor L2 ==
  Case-Ambient Insulated : fl_lib/Thermal/Thermal Elements/Perfect Insulator  T_specify=off  T_priority=None  T=0 K  T_nominal_specify=off  T_nominal_value=1  T_nominal_unit=K
  Iron Stack-Case Conductance : fl_lib/Thermal/Thermal Elements/Conductive Heat Transfer  thermal_type=foundation.enum.ConstantVariableTabulated.Constant  wall_geometry=foundation.enum.ConductionWallGeometry.Planar  area=4350 cm^2  thickness=1 cm  d_in=0.05 m  d_out=0.1 m  L=1 m  th_cond_min=10 W/(K*m)  th_cond=80.2 W/(m*K)  th_cond_TLU=[413, 401, 392, 383, 371, 357, 342] W/(K*m)  temp_TLU=[200, 273, 400, 600, 800, 1000, 1200] K  T_specify=off  T_priority=None  T=0 K  T_nominal_specify=off  T_nominal_value=1  T_nominal_unit=K  Q_specify=off  Q_priority=None  Q=0 W  Q_nominal_specify=off  Q_nominal_value=1  Q_nominal_unit=W
  Motor Case Thermal Mass : fl_lib/Thermal/Thermal Elements/Thermal Mass  mass_type=foundation.enum.constant_variable.constant  mass=5 kg  sp_heat=903 J/kg/K  mass_min=1e-6 kg  num_ports=foundation.enum.numPorts2.one  m_specify=off  m_priority=High  m=1 kg  m_nominal_specify=off  m_nominal_value=1  m_nominal_unit=kg  T_specify=off  T_priority=High  T=300 K  T_nominal_specify=off  T_nominal_value=1  T_nominal_unit=K  Q_specify=off  Q_priority=None  Q=0 W  Q_nominal_specify=off  Q_nominal_value=1  Q_nominal_unit=W
  Stator Iron Thermal Mass : fl_lib/Thermal/Thermal Elements/Thermal Mass  mass_type=foundation.enum.constant_variable.constant  mass=5 kg  sp_heat=447 J/kg/K  mass_min=1e-6 kg  num_ports=foundation.enum.numPorts2.one  m_specify=off  m_priority=High  m=1 kg  m_nominal_specify=off  m_nominal_value=1  m_nominal_unit=kg  T_specify=off  T_priority=High  T=300 K  T_nominal_specify=off  T_nominal_value=1  T_nominal_unit=K  Q_specify=off  Q_priority=None  Q=0 W  Q_nominal_specify=off  Q_nominal_value=1  Q_nominal_unit=W
  Winding Conductance : fl_lib/Thermal/Thermal Elements/Conductive Heat Transfer  thermal_type=foundation.enum.ConstantVariableTabulated.Constant  wall_geometry=foundation.enum.ConductionWallGeometry.Planar  area=250.2 cm^2  thickness=1 cm  d_in=0.05 m  d_out=0.1 m  L=1 m  th_cond_min=10 W/(K*m)  th_cond=401 W/(m*K)  th_cond_TLU=[413, 401, 392, 383, 371, 357, 342] W/(K*m)  temp_TLU=[200, 273, 400, 600, 800, 1000, 1200] K  T_specify=off  T_priority=None  T=0 K  T_nominal_specify=off  T_nominal_value=1  T_nominal_unit=K  Q_specify=off  Q_priority=None  Q=0 W  Q_nominal_specify=off  Q_nominal_value=1  Q_nominal_unit=W
  Winding Thermal Mass : fl_lib/Thermal/Thermal Elements/Thermal Mass  mass_type=foundation.enum.constant_variable.constant  mass=5 kg  sp_heat=385 J/kg/K  mass_min=1e-6 kg  num_ports=foundation.enum.numPorts2.one  m_specify=off  m_priority=High  m=1 kg  m_nominal_specify=off  m_nominal_value=1  m_nominal_unit=kg  T_specify=off  T_priority=High  T=300 K  T_nominal_specify=off  T_nominal_value=1  T_nominal_unit=K  Q_specify=off  Q_priority=None  Q=0 W  Q_nominal_specify=off  Q_nominal_value=1  Q_nominal_unit=W
  Winding-Iron Conductance : fl_lib/Thermal/Thermal Elements/Conductive Heat Transfer  thermal_type=foundation.enum.ConstantVariableTabulated.Constant  wall_geometry=foundation.enum.ConductionWallGeometry.Planar  area=250 cm^2  thickness=1 cm  d_in=0.05 m  d_out=0.1 m  L=1 m  th_cond_min=10 W/(K*m)  th_cond=360 W/(m*K)  th_cond_TLU=[413, 401, 392, 383, 371, 357, 342] W/(K*m)  temp_TLU=[200, 273, 400, 600, 800, 1000, 1200] K  T_specify=off  T_priority=None  T=0 K  T_nominal_specify=off  T_nominal_value=1  T_nominal_unit=K  Q_specify=off  Q_priority=None  Q=0 W  Q_nominal_specify=off  Q_nominal_value=1  Q_nominal_unit=W
  A : PMIOPort  Side=Left
  B : PMIOPort  Port=2  Side=Right
  connections:
  Winding Conductance/RConn1 -- A/RConn1
  B/RConn1 -- Winding-Iron Conductance/RConn1 -- Iron Stack-Case Conductance/LConn1 -- Stator Iron Thermal Mass/LConn1
  Case-Ambient Insulated/LConn1 -- Iron Stack-Case Conductance/RConn1 -- Motor Case Thermal Mass/LConn1
  Winding Thermal Mass/LConn1 -- Winding Conductance/LConn1 -- Winding-Iron Conductance/LConn1

== system sm_car_/Vehicle/Vehicle/Powertrain/Power/Electric L2 R2/Thermal/Liquid Loop1/Thermal Circuit Motor R2 ==
  Case-Ambient Insulated : fl_lib/Thermal/Thermal Elements/Perfect Insulator  T_specify=off  T_priority=None  T=0 K  T_nominal_specify=off  T_nominal_value=1  T_nominal_unit=K
  Iron Stack-Case Conductance : fl_lib/Thermal/Thermal Elements/Conductive Heat Transfer  thermal_type=foundation.enum.ConstantVariableTabulated.Constant  wall_geometry=foundation.enum.ConductionWallGeometry.Planar  area=4350 cm^2  thickness=1 cm  d_in=0.05 m  d_out=0.1 m  L=1 m  th_cond_min=10 W/(K*m)  th_cond=80.2 W/(m*K)  th_cond_TLU=[413, 401, 392, 383, 371, 357, 342] W/(K*m)  temp_TLU=[200, 273, 400, 600, 800, 1000, 1200] K  T_specify=off  T_priority=None  T=0 K  T_nominal_specify=off  T_nominal_value=1  T_nominal_unit=K  Q_specify=off  Q_priority=None  Q=0 W  Q_nominal_specify=off  Q_nominal_value=1  Q_nominal_unit=W
  Motor Case Thermal Mass : fl_lib/Thermal/Thermal Elements/Thermal Mass  mass_type=foundation.enum.constant_variable.constant  mass=5 kg  sp_heat=903 J/kg/K  mass_min=1e-6 kg  num_ports=foundation.enum.numPorts2.one  m_specify=off  m_priority=High  m=1 kg  m_nominal_specify=off  m_nominal_value=1  m_nominal_unit=kg  T_specify=off  T_priority=High  T=300 K  T_nominal_specify=off  T_nominal_value=1  T_nominal_unit=K  Q_specify=off  Q_priority=None  Q=0 W  Q_nominal_specify=off  Q_nominal_value=1  Q_nominal_unit=W
  Stator Iron Thermal Mass : fl_lib/Thermal/Thermal Elements/Thermal Mass  mass_type=foundation.enum.constant_variable.constant  mass=5 kg  sp_heat=447 J/kg/K  mass_min=1e-6 kg  num_ports=foundation.enum.numPorts2.one  m_specify=off  m_priority=High  m=1 kg  m_nominal_specify=off  m_nominal_value=1  m_nominal_unit=kg  T_specify=off  T_priority=High  T=300 K  T_nominal_specify=off  T_nominal_value=1  T_nominal_unit=K  Q_specify=off  Q_priority=None  Q=0 W  Q_nominal_specify=off  Q_nominal_value=1  Q_nominal_unit=W
  Winding Conductance : fl_lib/Thermal/Thermal Elements/Conductive Heat Transfer  thermal_type=foundation.enum.ConstantVariableTabulated.Constant  wall_geometry=foundation.enum.ConductionWallGeometry.Planar  area=250.2 cm^2  thickness=1 cm  d_in=0.05 m  d_out=0.1 m  L=1 m  th_cond_min=10 W/(K*m)  th_cond=401 W/(m*K)  th_cond_TLU=[413, 401, 392, 383, 371, 357, 342] W/(K*m)  temp_TLU=[200, 273, 400, 600, 800, 1000, 1200] K  T_specify=off  T_priority=None  T=0 K  T_nominal_specify=off  T_nominal_value=1  T_nominal_unit=K  Q_specify=off  Q_priority=None  Q=0 W  Q_nominal_specify=off  Q_nominal_value=1  Q_nominal_unit=W
  Winding Thermal Mass : fl_lib/Thermal/Thermal Elements/Thermal Mass  mass_type=foundation.enum.constant_variable.constant  mass=5 kg  sp_heat=385 J/kg/K  mass_min=1e-6 kg  num_ports=foundation.enum.numPorts2.one  m_specify=off  m_priority=High  m=1 kg  m_nominal_specify=off  m_nominal_value=1  m_nominal_unit=kg  T_specify=off  T_priority=High  T=300 K  T_nominal_specify=off  T_nominal_value=1  T_nominal_unit=K  Q_specify=off  Q_priority=None  Q=0 W  Q_nominal_specify=off  Q_nominal_value=1  Q_nominal_unit=W
  Winding-Iron Conductance : fl_lib/Thermal/Thermal Elements/Conductive Heat Transfer  thermal_type=foundation.enum.ConstantVariableTabulated.Constant  wall_geometry=foundation.enum.ConductionWallGeometry.Planar  area=250 cm^2  thickness=1 cm  d_in=0.05 m  d_out=0.1 m  L=1 m  th_cond_min=10 W/(K*m)  th_cond=360 W/(m*K)  th_cond_TLU=[413, 401, 392, 383, 371, 357, 342] W/(K*m)  temp_TLU=[200, 273, 400, 600, 800, 1000, 1200] K  T_specify=off  T_priority=None  T=0 K  T_nominal_specify=off  T_nominal_value=1  T_nominal_unit=K  Q_specify=off  Q_priority=None  Q=0 W  Q_nominal_specify=off  Q_nominal_value=1  Q_nominal_unit=W
  A : PMIOPort  Side=Left
  B : PMIOPort  Port=2  Side=Right
  connections:
  Winding Conductance/RConn1 -- A/RConn1
  B/RConn1 -- Winding-Iron Conductance/RConn1 -- Iron Stack-Case Conductance/LConn1 -- Stator Iron Thermal Mass/LConn1
  Case-Ambient Insulated/LConn1 -- Iron Stack-Case Conductance/RConn1 -- Motor Case Thermal Mass/LConn1
  Winding Thermal Mass/LConn1 -- Winding Conductance/LConn1 -- Winding-Iron Conductance/LConn1

== stateflow chart sm_car_/Controller/TrqVec 4Motor/Brake Control/ABS/Valve Control L2/Logic ==
  state Inactive
    entry:
    Mod_State = 1;
    Mod_Dur = 10;
  state Initial_Release
    entry:
    Mod_State = 2;
    Mod_Dur = 10;
  state Initial_Apply
    entry:
    Mod_State = 1;
    Mod_Dur = 6;
  state Release
    entry:
    Mod_State = 2;
    Mod_Dur = 6;
  state Apply
    entry:
    Mod_State = 1;
    Mod_Dur = 2;
  state Hold
    entry:
    Mod_State = 0;
    Mod_Dur = 6;
  (default) -> Inactive
  Apply -> Inactive [order 2] : [vSpdEst <0.1]
  Release -> Inactive [order 2] : [vSpdEst <0.1]
  Inactive -> Initial_Release : [Slip>0.5]
  Initial_Release -> Initial_Apply : [Slip<0.1]
  Release -> Initial_Apply [order 1] : [Slip <0.05]
  Initial_Apply -> Hold [order 2] : [Slip>0.1]
  Initial_Apply -> Apply [order 1] : [after(10,msec)]
  Hold -> Release [order 2] : [Slip > 0.25]
  Hold -> Apply [order 1] : [after(40,msec)]
  Apply -> Hold [order 1] : [Slip > 0.1]
  data: Slip input; Mod_State output; Mod_Dur output; vSpdEst input

== stateflow chart sm_car_/Controller/TrqVec 4Motor/Brake Control/ABS/Valve Control R1/Logic ==
  state Inactive
    entry:
    Mod_State = 1;
    Mod_Dur = 10;
  state Initial_Release
    entry:
    Mod_State = 2;
    Mod_Dur = 10;
  state Initial_Apply
    entry:
    Mod_State = 1;
    Mod_Dur = 6;
  state Release
    entry:
    Mod_State = 2;
    Mod_Dur = 6;
  state Apply
    entry:
    Mod_State = 1;
    Mod_Dur = 2;
  state Hold
    entry:
    Mod_State = 0;
    Mod_Dur = 6;
  (default) -> Inactive
  Apply -> Inactive [order 2] : [vSpdEst <0.1]
  Release -> Inactive [order 2] : [vSpdEst <0.1]
  Inactive -> Initial_Release : [Slip>0.5]
  Initial_Release -> Initial_Apply : [Slip<0.1]
  Release -> Initial_Apply [order 1] : [Slip <0.05]
  Initial_Apply -> Hold [order 2] : [Slip>0.1]
  Initial_Apply -> Apply [order 1] : [after(10,msec)]
  Hold -> Release [order 2] : [Slip > 0.25]
  Hold -> Apply [order 1] : [after(40,msec)]
  Apply -> Hold [order 1] : [Slip > 0.1]
  data: Slip input; Mod_State output; Mod_Dur output; vSpdEst input

== stateflow chart sm_car_/Controller/TrqVec 4Motor/Brake Control/ABS/Valve Control R2/Logic ==
  state Inactive
    entry:
    Mod_State = 1;
    Mod_Dur = 10;
  state Initial_Release
    entry:
    Mod_State = 2;
    Mod_Dur = 10;
  state Initial_Apply
    entry:
    Mod_State = 1;
    Mod_Dur = 6;
  state Release
    entry:
    Mod_State = 2;
    Mod_Dur = 6;
  state Apply
    entry:
    Mod_State = 1;
    Mod_Dur = 2;
  state Hold
    entry:
    Mod_State = 0;
    Mod_Dur = 6;
  (default) -> Inactive
  Apply -> Inactive [order 2] : [vSpdEst <0.1]
  Release -> Inactive [order 2] : [vSpdEst <0.1]
  Inactive -> Initial_Release : [Slip>0.5]
  Initial_Release -> Initial_Apply : [Slip<0.1]
  Release -> Initial_Apply [order 1] : [Slip <0.05]
  Initial_Apply -> Hold [order 2] : [Slip>0.1]
  Initial_Apply -> Apply [order 1] : [after(10,msec)]
  Hold -> Release [order 2] : [Slip > 0.25]
  Hold -> Apply [order 1] : [after(40,msec)]
  Apply -> Hold [order 1] : [Slip > 0.1]
  data: Slip input; Mod_State output; Mod_Dur output; vSpdEst input
